simulink model "SYSTEM_MODEL"  (R2024a)
settings: Solver=ode45  StartTime=0.0  StopTime=0.5  RelTol=1e-3
values from neighbouring files (symbols this model uses):
  Cf = x*Cb    (= 0.000348151438014)    [parameters.m]
  Fsw = 10e3    (= 10000)    [parameters.m]
  kii = 219.7931    [parameters.m]
  kiv = 645.1962    [parameters.m]
  kpi = 4.9973    [parameters.m]
  kpv = 2.0537    [parameters.m]
  L = Vdc/(8*Fsw*I_ripple)    [parameters.m]
  Lf = L*r    [parameters.m]
  Lt = L+Lf    [parameters.m]
  R = 0.004    [parameters.m]
  Rf = 0.001    [parameters.m]
  Vdc = 800    [parameters.m]
undefined symbols (not defined in the file or in its folder): Ion, Lithium
libraries: spsIGBTDiodeLib x7, spsSeriesRLCBranchLib x5, slpidlib x5, spsCurrentMeasurementLib x3, spsVoltageMeasurementLib x3, spsThreePhaseSeriesRLCBranchLib x3, spsabctodq0Lib x2, simulink x1, spsIGBTLib x1, spsPWMGeneratorDCDCLib x1, spsBatteryLib x1, spsGroundLib x1
settings Model: Creator=devashishraj  LastModifiedBy=loran
settings DebuggingCC: UnconnectedInputMsg=warning  UnconnectedOutputMsg=warning  UnconnectedLineMsg=warning
settings ModelReferenceCC: EnableRefExpFcnMdlSchedulingChecks=on
settings RTWCC: GPUComputeCapability=3.5  DLArmComputeVersion=19.05

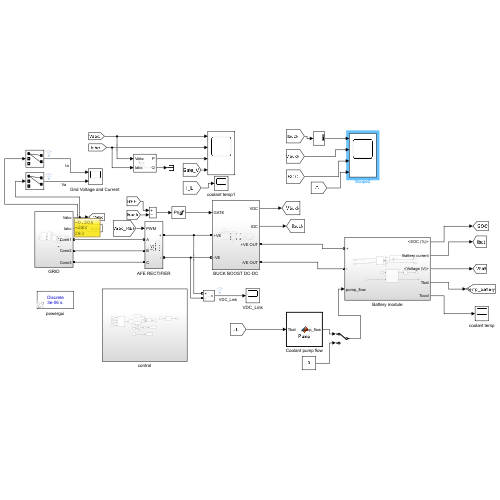
[thumbnail: Simulink's stored preview of the top-level diagram]
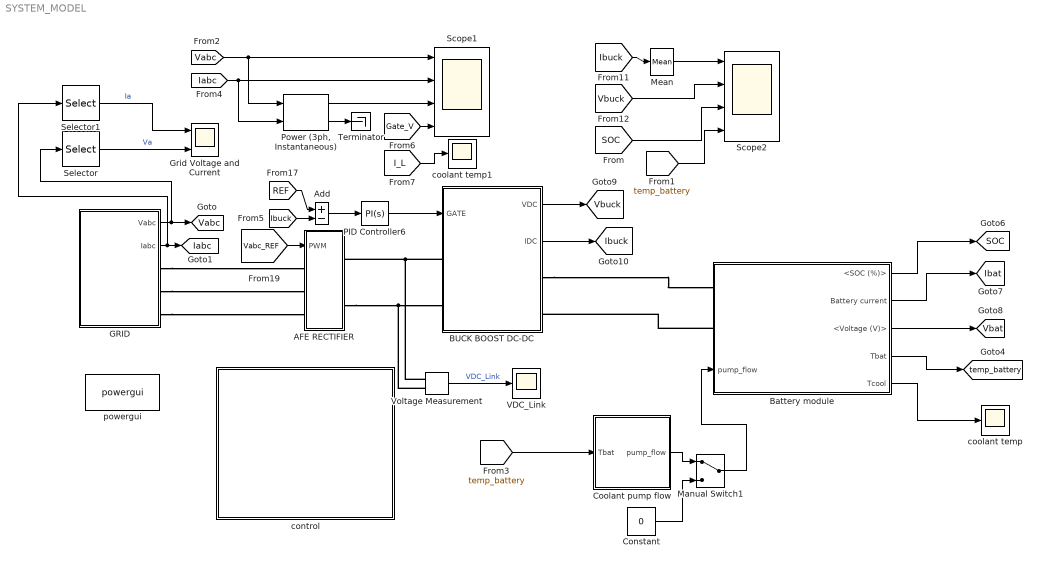
== system SYSTEM_MODEL ==
  AFE RECTIFIER : Subsystem
  Add : Sum  Inputs=+-
  BUCK BOOST DC-DC : Subsystem
  Battery module : Subsystem
      settings: PortSchema="{\"entries\":[{\"content\":{\"sides\":[{\"content\":{\"connectorIds\":[\"LConn1\",\"LConn2\",\"In1\"]},\"type\":\"ConnectorPlacement.EquallySpacedRectSide\",\"uuid\":\"b9a7e7ab-cfc6-4f27-ac3f-4a3ea86e3158\"},{\"content\":{\"connectorIds\":[\"Out1\",\"Out2\",\"Out3\",\"Out4\",\"Out5\"],\"side\":\"RIGHT\"},\"type\":\"ConnectorPlacement.EquallySpacedRectSide\",\"uuid\":\"900f3018-bf12-407b-85a8-bc4a87dc546d\"},{\"content\":{\"side\":\"TOP\"},\"type\":\"ConnectorPlacement.EquallySpacedRectSide\",\"uuid\":\"2d743f8c-64eb-4470-8afd-3ba3a990ea7c\"},{\"content\":{\"side\":\"BOTTOM\"},\"type\":\"ConnectorPlacement.EquallySpacedRectSide\",\"uuid\":\"3e69f90f-b07e-44a2-b438-8ead40159241\"}]},\"type\":\"ConnectorPlacement.EquallySpacedConnector\",\"uuid\":\"2127e1cc-c587-4944-bbda-621e2cf85e2c\"}],\"packageUris\":[\"http://schema.mathworks.com/mf0/Connector/R2020b\"],\"version\":\"1.0\"}"
  Constant : Constant  Value=0
  Coolant pump flow : MATLAB Function  TreatAsAtomicUnit=on
  GRID : Subsystem
  "Grid Voltage and Current " : Scope  NumInputPorts=2
  Manual Switch1 : ManualSwitch
  Mean : spsMeanLib/Mean  Freq=100  Vinit=0  Ts=0
  PID Controller6 : slpidlib/PID Controller  Controller=PI  Form=Parallel  TimeDomain=Continuous-time  UseExternalTs=off  SampleTime=-1  IntegratorMethod=Forward Euler  FilterMethod=Forward Euler  ControllerParametersSource=internal  P=800.07973079426302e-05  I=3.0202336655835159303  UseKiTs=off  D=0  UseExternalDerivativeSource=off  N=100  UseFilter=on  TunerSelectOption=Transfer Function Based (PID Tuner App)  ZeroCross=off  InitialConditionSource=internal  InitialConditionForIntegrator=0  InitialConditionForFilter=0  DifferentiatorICPrevScaledInput=0  ExternalReset=none  TrackingMode=off  Kt=1  LimitOutput=on  SatLimitsSource=internal  UpperSaturationLimit=0.47  LowerSaturationLimit=0  LinearizeAsGain=on  AntiWindupMode=clamping  Kb=1  LimitIntegrator=off  UpperIntegratorSaturationLimit=inf  LowerIntegratorSaturationLimit=-inf  POutMin=[]  POutMax=[]  IOutMin=[]  IOutMax=[]  DOutMin=[]  DOutMax=[]  NOutMin=[]  NOutMax=[]  SumOutMin=[]  SumOutMax=[]  SaturationOutMin=[]  SaturationOutMax=[]  PParamMin=[]  PParamMax=[]  IParamMin=[]  IParamMax=[]  DParamMin=[]  DParamMax=[]  NParamMin=[]  NParamMax=[]  KbParamMin=[]  KbParamMax=[]  KtParamMin=[]  KtParamMax=[]  KbOutMin=[]  KbOutMax=[]  KtOutMin=[]  KtOutMax=[]  IntegratorOutMin=[]  IntegratorOutMax=[]  FilterOutMin=[]  FilterOutMax=[]  SumI1OutMin=[]  SumI1OutMax=[]  SumI2OutMin=[]  SumI2OutMax=[]  SumI3OutMin=[]  SumI3OutMax=[]  SumI4OutMin=[]  SumI4OutMax=[]  SumDOutMin=[]  SumDOutMax=[]  DifferentiatorOutMin=[]  DifferentiatorOutMax=[]  FilterDiffOutCoefMin=[]  FilterDiffOutCoefMax=[]  ReciprocalOutMin=[]  ReciprocalOutMax=[]  SumDenOutMin=[]  SumDenOutMax=[]  SumNumOutMin=[]  SumNumOutMax=[]  DivideOutMin=[]  DivideOutMax=[]  UdiffTsProdOutMin=[]  UdiffTsProdOutMax=[]  NTsProdOutMin=[]  NTsProdOutMax=[]  UintegralTsProdOutMin=[]  UintegralTsProdOutMax=[]  UngainTsProdOutMin=[]  UngainTsProdOutMax=[]  ClampingZeroOutDataTypeStr=Inherit: Inherit via back propagation  ClampingZeroOutMin=[]  ClampingZeroOutMax=[]  FilterDenConstantOutDataTypeStr=Inherit: Inherit via back propagation  FilterDenConstantOutMin=[]  FilterDenConstantOutMax=[]  PCopyOutDataTypeStr=Inherit: Inherit via back propagation  PCopyOutMin=[]  PCopyOutMax=[]  NCopyOutDataTypeStr=Inherit: Inherit via back propagation  NCopyOutMin=[]  NCopyOutMax=[]  IntegratorContinuousStateAttributes=''  IntegratorStateMustResolveToSignalObject=off  IntegratorRTWStateStorageClass=Auto  FilterContinuousStateAttributes=''  FilterStateMustResolveToSignalObject=off  FilterRTWStateStorageClass=Auto  ParallelPVariant=InternalParameters  IdealPVariant=Disabled  IVariant=InternalParameters  DVariant=Disabled  IntegratorVariant=Continuous  SatVariant=Enabled  AWVariant=ContClampingParallel  PCopyVariant=Disabled  TRVariant=Disabled  FdbkBlocksVariant=Forward  IdealPFdbkVariant=Disabled  SatFdbkVariant=Disabled  DerivativeFilterVariant=Disabled  NVariant=Disabled  NCopyVariant=Disabled_SignalSpec  FilterICVariant=Disabled  IntegratorICVariant=InternalICs  ExternalResetVariant=Disabled  TRSumVariant=Passthrough  SumFdbkVariant=Disabled  SumVariant=Sum_PI  TsampFilterVariant=InternalTs  TsampNgainVariant=Passthrough  TsampIntegralVariant=Disabled_SignalSpec  ExternalSaturationOutDataTypeStr=Inherit: Same as second input  DerivativeSourceVariant=Disabled
  "Power (3ph, Instantaneous)" : spsPower3phInstantaneousLib/Power (3ph, Instantaneous)
  Scope1 : Scope  NumInputPorts=4
  Scope2 : Scope  NumInputPorts=4
  Selector : Selector  InputPortWidth=3  IndexOptions=Index vector (dialog)  Indices=[1 1]  OutputSizes=1
  Selector1 : Selector  InputPortWidth=3  IndexOptions=Index vector (dialog)  Indices=[1 1]  OutputSizes=1
  Terminator : Terminator
  VDC_Link : Scope
  Voltage Measurement : spsVoltageMeasurementLib/Voltage Measurement  PhasorSimulation=off  OutputType=Complex  PSBequivalent=0
  control : Subsystem
  coolant temp : Scope
  coolant temp1 : Scope
  powergui : spspowerguiLib/powergui  Priority=1  SimulationMode=Discrete  SampleTime=3e-6  frequency=60  Iterations=50  frequencyindice=0  Pbase=100e6  ErrMax=1e-4  UnitsV=kV  UnitsW=MW  buscounter=0  FunctionMessages=off  echomessages=off  EnableUseOfTLC=off  CurrentSourceSwitches=off  DisableSnubberDevices=off  DisableRonSwitches=off  DisableVfSwitches=off  DisplayEquations=off  AutomaticDiscreteSolvers=off  SolverType=Tustin/Backward Euler (TBE)  Interpol=off  ExternalGateDelay=off  methode=off  Ts=100  x0status=blocks  SPID=on  SwTol=0  HookPort=off  NonlinearTolerance=1e-4  nMaxIteration=100  ContinueOnMaxIteration=off  RestoreLinks=warning  ResistiveCurrentMeasurement=off  Frange=[0:2:500]  Ylog=off  Xlog=on  ShowGrid=off  save=off  variable=ZData  structure=0  ZoomFFT=off  StartTime=0.0  cycles=1  DisplayStyle=1  fundamental=60  FreqAxis=off  MaxFrequency=1000  frequencyindicesteady=1  RmsSteady=1  display=off
  tag scope: Iabc=global, Ibat=global, Ibuck=global, SOC=global, Vabc=global, Vbat=global, Vbuck=global, temp_battery=global
  wires:
  GRID/1(Vabc) -> Selector/1, [Vabc]
  GRID/2(Iabc) -> Selector1/1, [Iabc]
  [Ibuck] -> Add/2
  Add/1 -> PID Controller6/1
  [Ibuck] -> Mean/1
  [SOC] -> Scope2/3
  [REF] -> Add/1
  [Vabc_REF] -> AFE RECTIFIER/1(PWM)
  PID Controller6/1 -> BUCK BOOST DC-DC/1(GATE)
  BUCK BOOST DC-DC/1(VDC) -> [Vbuck]
  BUCK BOOST DC-DC/2(IDC) -> [Ibuck]
  [Vbuck] -> Scope2/2
  Mean/1 -> Scope2/1
  [temp_battery] -> Scope2/4
  Coolant pump flow/1(pump_flow) -> Manual Switch1/1
  Battery module/1(<SOC (%)>) -> [SOC]
  Battery module/2(Battery current) -> [Ibat]
  Battery module/3(<Voltage (V)>) -> [Vbat]
  Battery module/4(Tbat) -> [temp_battery]
  Battery module/5(Tcool) -> coolant temp/1
  Constant/1 -> Manual Switch1/2
  [temp_battery] -> Coolant pump flow/1(Tbat)
  Manual Switch1/1 -> Battery module/1(pump_flow)
  [Iabc] -> "Power (3ph, Instantaneous)"/2, Scope1/2
  [Vabc] -> "Power (3ph, Instantaneous)"/1, Scope1/1
  "Power (3ph, Instantaneous)"/1 -> Scope1/3
  [Gate_V] -> Scope1/4
  "Power (3ph, Instantaneous)"/2 -> Terminator/1
  [I_L] -> coolant temp1/1
  Selector1/1 -> "Grid Voltage and Current "/1  "Ia"
  Selector/1 -> "Grid Voltage and Current "/2  "Va"
  Voltage Measurement/1 -> VDC_Link/1  "VDC_Link"
  connections:
  GRID/RConn1 -- AFE RECTIFIER/LConn1
  GRID/RConn2 -- AFE RECTIFIER/LConn2
  GRID/RConn3 -- AFE RECTIFIER/LConn3
  BUCK BOOST DC-DC/LConn1 -- Voltage Measurement/LConn1 -- AFE RECTIFIER/RConn1
  AFE RECTIFIER/RConn2 -- Voltage Measurement/LConn2 -- BUCK BOOST DC-DC/LConn2
  BUCK BOOST DC-DC/RConn1 -- Battery module/LConn1
  Battery module/LConn2 -- BUCK BOOST DC-DC/RConn2

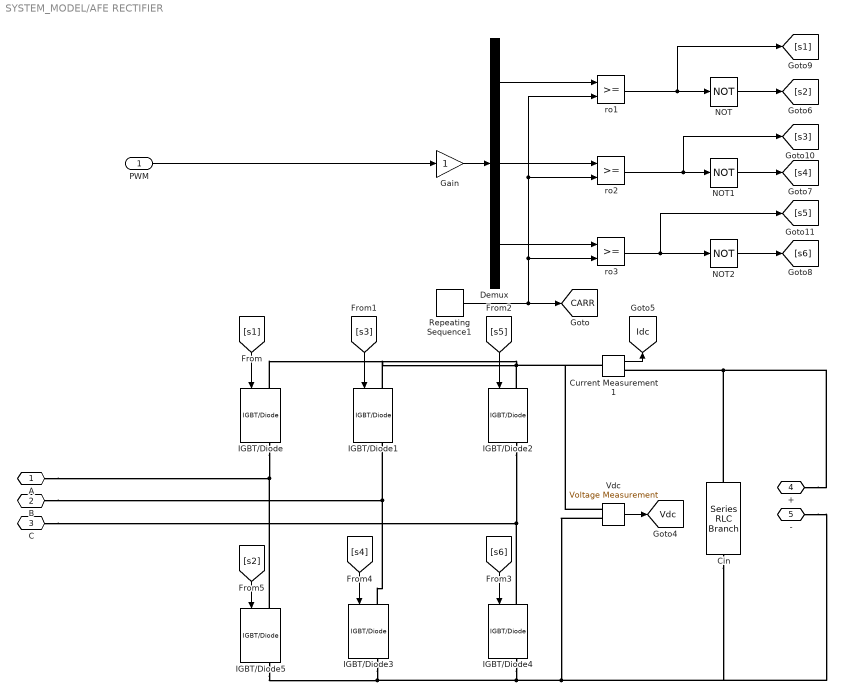
== system SYSTEM_MODEL/AFE RECTIFIER ==
  PWM : Inport
  Cin : spsSeriesRLCBranchLib/Series RLC Branch  LConnTagsString=__new0  RConnTagsString=__new0  BranchType=C  Resistance=1  Inductance=1e-3  SetiL0=off  InitialCurrent=0  Capacitance=1000e-6  Setx0=off  InitialVoltage=600  Measurements=None
  Current Measurement1 : spsCurrentMeasurementLib/Current Measurement  PhasorSimulation=off  OutputType=Complex  PSBequivalent=0
  Demux : Demux  Outputs=3
  Gain : Gain
  IGBT/Diode{,1..5} (6 alike) : spsIGBTDiodeLib/IGBT//Diode  Ron=1e-3  Rs=1e5  Cs=inf  Measurements=on
  NOT : Logic  Operator=NOT  IconShape=distinctive  AllPortsSameDT=off  OutDataTypeStr=boolean
  NOT1 : Logic  Operator=NOT  IconShape=distinctive  AllPortsSameDT=off  OutDataTypeStr=boolean
  NOT2 : Logic  Operator=NOT  IconShape=distinctive  AllPortsSameDT=off  OutDataTypeStr=boolean
  Repeating Sequence1 : simulink/Sources/Repeating Sequence  rep_seq_t="[0  1/(2*Fsw) 1/Fsw ]"  rep_seq_y=[-1000 1000 -1000]
  Vdc : spsVoltageMeasurementLib/Voltage Measurement  PhasorSimulation=off  OutputType=Complex  PSBequivalent=0
  ro1 : RelationalOperator  OutDataTypeStr=boolean  RndMeth=Simplest  InputSameDT=off
  ro2 : RelationalOperator  OutDataTypeStr=boolean  RndMeth=Simplest  InputSameDT=off
  ro3 : RelationalOperator  OutDataTypeStr=boolean  RndMeth=Simplest  InputSameDT=off
  A : PMIOPort  Side=Left
  B : PMIOPort  Port=2  Side=Left
  C : PMIOPort  Port=3  Side=Left
  + : PMIOPort  Port=4  Side=Right
  - : PMIOPort  Port=5  Side=Right
  tag scope: CARR=global, Idc=global, Vdc=global
  wires:
  NOT2/1 -> [s6]
  Demux/2 -> ro2/1
  PWM/1 -> Gain/1
  [s3] -> IGBT/Diode1/1
  Current Measurement1/1 -> [Idc]
  [s1] -> IGBT/Diode/1
  [s4] -> IGBT/Diode3/1
  Gain/1 -> Demux/1
  Demux/1 -> ro1/1
  [s2] -> IGBT/Diode5/1
  [s5] -> IGBT/Diode2/1
  ro1/1 -> [s1], NOT/1
  ro2/1 -> [s3], NOT1/1
  Demux/3 -> ro3/1
  NOT1/1 -> [s4]
  NOT/1 -> [s2]
  [s6] -> IGBT/Diode4/1
  Vdc/1 -> [Vdc]
  ro3/1 -> [s5], NOT2/1
  Repeating Sequence1/1 -> ro3/2, ro2/2, ro1/2, [CARR]
  connections:
  C/RConn1 -- IGBT/Diode4/LConn1 -- IGBT/Diode2/RConn1
  -/RConn1 -- Cin/RConn1 -- Vdc/LConn2 -- IGBT/Diode5/RConn1 -- IGBT/Diode3/RConn1 -- IGBT/Diode4/RConn1
  Cin/LConn1 -- +/RConn1 -- Current Measurement1/RConn1
  Vdc/LConn1 -- Current Measurement1/LConn1 -- IGBT/Diode2/LConn1 -- IGBT/Diode/LConn1 -- IGBT/Diode1/LConn1
  B/RConn1 -- IGBT/Diode3/LConn1 -- IGBT/Diode1/RConn1
  A/RConn1 -- IGBT/Diode5/LConn1 -- IGBT/Diode/RConn1

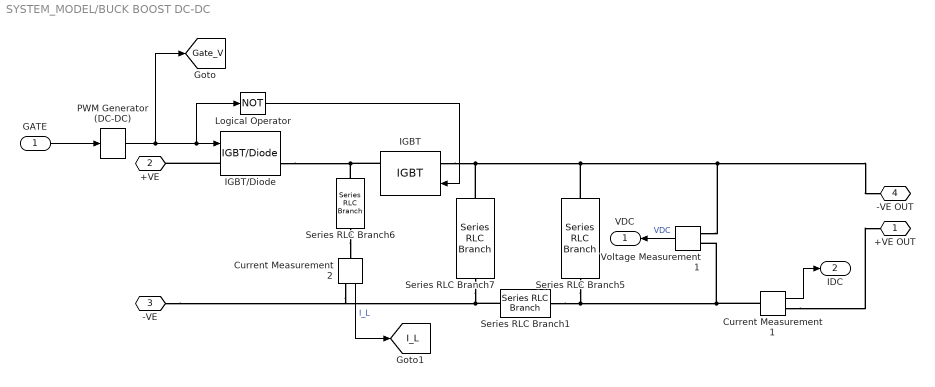
== system SYSTEM_MODEL/BUCK BOOST DC-DC ==
  GATE : Inport
  Current Measurement1 : spsCurrentMeasurementLib/Current Measurement  PhasorSimulation=off  OutputType=Complex  PSBequivalent=0
  Current Measurement2 : spsCurrentMeasurementLib/Current Measurement  PhasorSimulation=off  OutputType=Complex  PSBequivalent=0
  IGBT : spsIGBTLib/IGBT  Ron=0.001  Lon=0  Vf=1  Tf=1e-6  Tt=2e-6  IC=0  Rs=1e5  Cs=inf  Measurements=on
  IGBT/Diode : spsIGBTDiodeLib/IGBT//Diode  Ron=1e-3  Rs=1e5  Cs=inf  Measurements=on
  Logical Operator : Logic  Operator=NOT  AllPortsSameDT=off  OutDataTypeStr=boolean
  PWM Generator (DC-DC) : spsPWMGeneratorDCDCLib/PWM Generator (DC-DC)  Fsw=100e3  Ts=0
  Series RLC Branch1 : spsSeriesRLCBranchLib/Series RLC Branch  LConnTagsString=__new0  RConnTagsString=__new0  BranchType=L  Resistance=1  Inductance=3e-3  SetiL0=on  InitialCurrent=0  Capacitance=1e-6  Setx0=off  InitialVoltage=0  Measurements=Branch current
  Series RLC Branch5 : spsSeriesRLCBranchLib/Series RLC Branch  LConnTagsString=__new0  RConnTagsString=__new0  BranchType=C  Resistance=1  Inductance=1e-3  SetiL0=off  InitialCurrent=0  Capacitance=500e-6  Setx0=on  InitialVoltage=0  Measurements=None
  Series RLC Branch6 : spsSeriesRLCBranchLib/Series RLC Branch  LConnTagsString=__new0  RConnTagsString=__new0  BranchType=L  Resistance=1  Inductance=36e-6  SetiL0=on  InitialCurrent=0  Capacitance=1e-6  Setx0=off  InitialVoltage=0  Measurements=Branch current
  Series RLC Branch7 : spsSeriesRLCBranchLib/Series RLC Branch  LConnTagsString=__new0  RConnTagsString=__new0  BranchType=C  Resistance=1  Inductance=1e-3  SetiL0=off  InitialCurrent=0  Capacitance=20e-6  Setx0=on  InitialVoltage=0  Measurements=None
  Voltage Measurement1 : spsVoltageMeasurementLib/Voltage Measurement  PhasorSimulation=off  OutputType=Complex  PSBequivalent=0
  +VE OUT : PMIOPort  Side=Right
  +VE : PMIOPort  Port=2  Side=Left
  -VE : PMIOPort  Port=3  Side=Left
  -VE OUT : PMIOPort  Port=4  Side=Right
  VDC : Outport
  IDC : Outport  Port=2
  tag scope: Gate_V=global, I_L=global
  wires:
  Logical Operator/1 -> IGBT/1
  Current Measurement1/1 -> IDC/1
  GATE/1 -> PWM Generator (DC-DC)/1
  PWM Generator (DC-DC)/1 -> [Gate_V], IGBT/Diode/1, Logical Operator/1
  Voltage Measurement1/1 -> VDC/1  "VDC"
  Current Measurement2/1 -> [I_L]  "I_L"
  connections:
  IGBT/LConn1 -- Series RLC Branch7/RConn1 -- Series RLC Branch5/RConn1 -- -VE OUT/RConn1 -- Voltage Measurement1/LConn2
  Series RLC Branch5/LConn1 -- Series RLC Branch1/RConn1 -- Voltage Measurement1/LConn1 -- Current Measurement1/LConn1
  Series RLC Branch1/LConn1 -- -VE/RConn1 -- Current Measurement2/RConn1 -- Series RLC Branch7/LConn1
  IGBT/RConn1 -- Series RLC Branch6/RConn1 -- IGBT/Diode/RConn1
  IGBT/Diode/LConn1 -- +VE/RConn1
  Current Measurement1/RConn1 -- +VE OUT/RConn1
  Series RLC Branch6/LConn1 -- Current Measurement2/LConn1

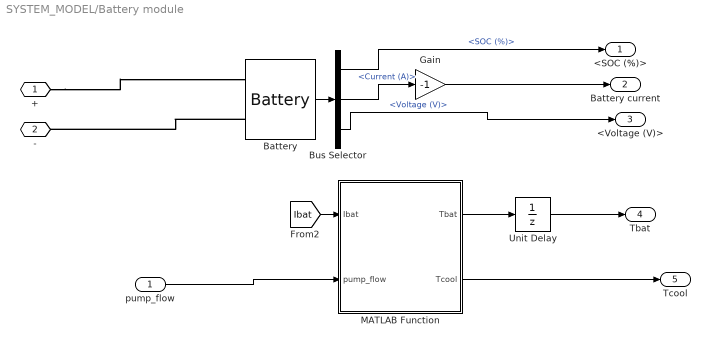
== system SYSTEM_MODEL/Battery module ==
  pump_flow : Inport
  Battery : spsBatteryLib/Battery  BatType=Lithium-Ion  ShowTempParam=off  ThermalPreset=no  ShowAgeParam=off  NomV=400  NomQ=250  SOC=20  Batt_Tr=1  PresetModel=on  MaxQ=250  MinV=300  FullV=465.5949  Dis_rate=108.6957  R=0.016  Normal_OP=226.087  expZone="[432.1543      12.28261]"  current=[6.5 13 32.5]  Units=Time  Tci=25  NomT=25  T2=20  MaxQ2=250  FullV2=400  Normal_OP2=440  expZone2=[450 250]  Rca=0.6  ti=2000  Dp=0  Neq0=0  Tsim=1e6  Ta1=25  Qeol=5.4*0.9  Reol=0.013333*1.2  Char_age=[2.3478, 3]  Dis_age=[2.3478, 10]  N1=1500  N2=10500  N3=1000  N4=1400  Ta2=45  N5=950
  Bus Selector : BusSelector  OutputSignals=SOC (%),Current (A),Voltage (V)
  Gain : Gain  Gain=-1
  MATLAB Function : MATLAB Function  TreatAsAtomicUnit=on
  Unit Delay : UnitDelay  SampleTime=-1  HasFrameUpgradeWarning=on
  + : PMIOPort  Side=Left
  - : PMIOPort  Port=2  Side=Left
  <SOC (%)> : Outport
  Battery current : Outport  Port=2
  <Voltage (V)> : Outport  Port=3
  Tbat : Outport  Port=4
  Tcool : Outport  Port=5
  wires:
  MATLAB Function/2(Tcool) -> Tcool/1
  Bus Selector/1 -> <SOC (%)>/1  "<SOC (%)>"
  Battery/1 -> Bus Selector/1
  [Ibat] -> MATLAB Function/1(Ibat)
  Bus Selector/2 -> Gain/1  "<Current (A)>"
  pump_flow/1 -> MATLAB Function/2(pump_flow)
  Bus Selector/3 -> <Voltage (V)>/1  "<Voltage (V)>"
  MATLAB Function/1(Tbat) -> Unit Delay/1
  Gain/1 -> Battery current/1
  Unit Delay/1 -> Tbat/1
  connections:
  Battery/LConn2 -- -/RConn1
  +/RConn1 -- Battery/LConn1

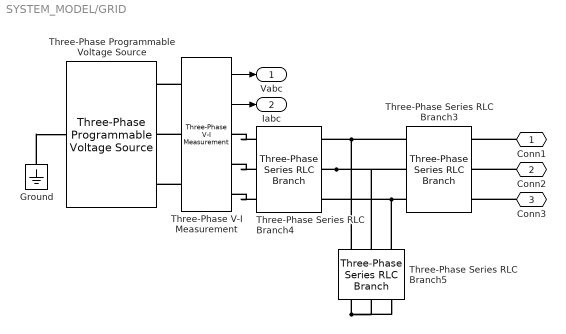
== system SYSTEM_MODEL/GRID ==
  Ground : spsGroundLib/Ground  LConnTagsString=a
  Three-Phase Programmable Voltage Source : spsThreePhaseProgrammableVoltageSourceLib/Three-Phase Programmable Voltage Source  PositiveSequence="[400  0 50]"  VariationEntity=None  VariationType=Table of time-amplitude pairs  VariationTypeAlt=Step  VariationStep=0.5  VariationRate=10  VariationMagnitude=0.3  VariationFrequency=2  VariationTiming=[1 2]  VariationPhaseA=off  Amplitudes=[1 0.8 1.2 1.0]  TimeValues=[0 0.1 0.15 0.2]  HarmonicGeneration=off  HarmonicA=[3 0.2 -25 0]  HarmonicB=[2 0.15 35 2]  Timing="[0.05  3]"  BusType=swing  Pref=0  Qref=0  Qmin=-inf  Qmax=inf
  Three-Phase Series RLC Branch3 : spsThreePhaseSeriesRLCBranchLib/Three-Phase Series RLC Branch  LConnTagsString=A|B|C  RConnTagsString=A|B|C  BranchType=RL  Resistance=R  Inductance=L  Capacitance=1e-6  Measurements=None
  Three-Phase Series RLC Branch4 : spsThreePhaseSeriesRLCBranchLib/Three-Phase Series RLC Branch  LConnTagsString=A|B|C  RConnTagsString=A|B|C  BranchType=RL  Resistance=Rf  Inductance=Lf  Capacitance=1e-6  Measurements=None
  Three-Phase Series RLC Branch5 : spsThreePhaseSeriesRLCBranchLib/Three-Phase Series RLC Branch  LConnTagsString=A|B|C  RConnTagsString=A|B|C  BranchType=RC  Resistance=2  Inductance=150e-6  Capacitance=Cf  Measurements=None
  Three-Phase V-I Measurement : spsThreePhaseVIMeasurementLib/Three-Phase V-I Measurement  VoltageMeasurement=phase-to-ground  SetLabelV=off  LabelV=Vabc  Vpu=off  VpuLL=off  CurrentMeasurement=yes  SetLabelI=off  LabelI=Iabc  Ipu=off  Pbase=100e6  Vbase=500e3  OutputType=Complex  PhasorSimulation=off  PSBequivalent=0
  Conn1 : PMIOPort  Side=Right
  Conn2 : PMIOPort  Port=2  Side=Right
  Conn3 : PMIOPort  Port=3  Side=Right
  Vabc : Outport
  Iabc : Outport  Port=2
  wires:
  Three-Phase V-I Measurement/1 -> Vabc/1
  Three-Phase V-I Measurement/2 -> Iabc/1
  connections:
  Three-Phase V-I Measurement/LConn1 -- Three-Phase Programmable Voltage Source/RConn1
  Three-Phase V-I Measurement/LConn3 -- Three-Phase Programmable Voltage Source/RConn3
  Three-Phase V-I Measurement/LConn2 -- Three-Phase Programmable Voltage Source/RConn2
  Ground/LConn1 -- Three-Phase Programmable Voltage Source/LConn1
  Three-Phase Series RLC Branch4/LConn2 -- Three-Phase Series RLC Branch5/LConn2 -- Three-Phase Series RLC Branch3/RConn2
  Three-Phase Series RLC Branch3/RConn3 -- Three-Phase Series RLC Branch4/LConn3 -- Three-Phase Series RLC Branch5/LConn3
  Three-Phase Series RLC Branch5/LConn1 -- Three-Phase Series RLC Branch4/LConn1 -- Three-Phase Series RLC Branch3/RConn1
  Three-Phase Series RLC Branch5/RConn1 -- Three-Phase Series RLC Branch5/RConn2 -- Three-Phase Series RLC Branch5/RConn3
  Conn3/RConn1 -- Three-Phase Series RLC Branch3/LConn3
  Conn1/RConn1 -- Three-Phase Series RLC Branch3/LConn1
  Conn2/RConn1 -- Three-Phase Series RLC Branch3/LConn2
  Three-Phase Series RLC Branch4/RConn1 -- Three-Phase V-I Measurement/RConn1
  Three-Phase Series RLC Branch4/RConn2 -- Three-Phase V-I Measurement/RConn2
  Three-Phase Series RLC Branch4/RConn3 -- Three-Phase V-I Measurement/RConn3

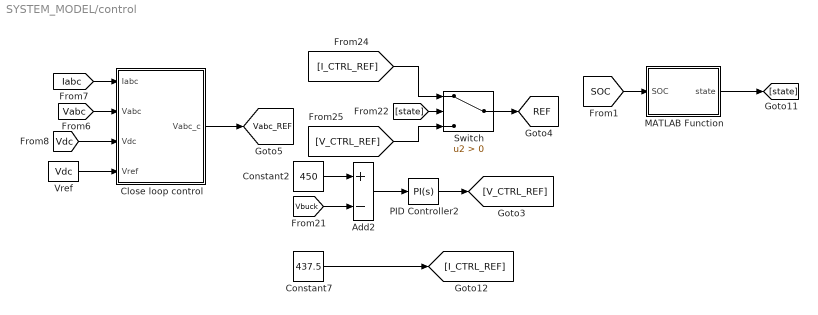
== system SYSTEM_MODEL/control ==
  Add2 : Sum  Inputs=+-
  Close loop control : Subsystem
  Constant2 : Constant  Value=450  SampleTime=2e-6
  Constant7 : Constant  Value=437.5  SampleTime=2e-6
  MATLAB Function : MATLAB Function  TreatAsAtomicUnit=on
  PID Controller2 : slpidlib/PID Controller  Controller=PI  Form=Parallel  TimeDomain=Continuous-time  UseExternalTs=off  SampleTime=-1  IntegratorMethod=Forward Euler  FilterMethod=Forward Euler  ControllerParametersSource=internal  P=0.75  I=50  UseKiTs=off  D=0  UseExternalDerivativeSource=off  N=100  UseFilter=on  TunerSelectOption=Transfer Function Based (PID Tuner App)  ZeroCross=off  InitialConditionSource=internal  InitialConditionForIntegrator=0  InitialConditionForFilter=0  DifferentiatorICPrevScaledInput=0  ExternalReset=none  TrackingMode=off  Kt=1  LimitOutput=on  SatLimitsSource=internal  UpperSaturationLimit=500  LowerSaturationLimit=0  LinearizeAsGain=on  AntiWindupMode=clamping  Kb=1  LimitIntegrator=off  UpperIntegratorSaturationLimit=inf  LowerIntegratorSaturationLimit=-inf  POutMin=[]  POutMax=[]  IOutMin=[]  IOutMax=[]  DOutMin=[]  DOutMax=[]  NOutMin=[]  NOutMax=[]  SumOutMin=[]  SumOutMax=[]  SaturationOutMin=[]  SaturationOutMax=[]  PParamMin=[]  PParamMax=[]  IParamMin=[]  IParamMax=[]  DParamMin=[]  DParamMax=[]  NParamMin=[]  NParamMax=[]  KbParamMin=[]  KbParamMax=[]  KtParamMin=[]  KtParamMax=[]  KbOutMin=[]  KbOutMax=[]  KtOutMin=[]  KtOutMax=[]  IntegratorOutMin=[]  IntegratorOutMax=[]  FilterOutMin=[]  FilterOutMax=[]  SumI1OutMin=[]  SumI1OutMax=[]  SumI2OutMin=[]  SumI2OutMax=[]  SumI3OutMin=[]  SumI3OutMax=[]  SumI4OutMin=[]  SumI4OutMax=[]  SumDOutMin=[]  SumDOutMax=[]  DifferentiatorOutMin=[]  DifferentiatorOutMax=[]  FilterDiffOutCoefMin=[]  FilterDiffOutCoefMax=[]  ReciprocalOutMin=[]  ReciprocalOutMax=[]  SumDenOutMin=[]  SumDenOutMax=[]  SumNumOutMin=[]  SumNumOutMax=[]  DivideOutMin=[]  DivideOutMax=[]  UdiffTsProdOutMin=[]  UdiffTsProdOutMax=[]  NTsProdOutMin=[]  NTsProdOutMax=[]  UintegralTsProdOutMin=[]  UintegralTsProdOutMax=[]  UngainTsProdOutMin=[]  UngainTsProdOutMax=[]  ClampingZeroOutDataTypeStr=Inherit: Inherit via back propagation  ClampingZeroOutMin=[]  ClampingZeroOutMax=[]  FilterDenConstantOutDataTypeStr=Inherit: Inherit via back propagation  FilterDenConstantOutMin=[]  FilterDenConstantOutMax=[]  PCopyOutDataTypeStr=Inherit: Inherit via back propagation  PCopyOutMin=[]  PCopyOutMax=[]  NCopyOutDataTypeStr=Inherit: Inherit via back propagation  NCopyOutMin=[]  NCopyOutMax=[]  IntegratorContinuousStateAttributes=''  IntegratorStateMustResolveToSignalObject=off  IntegratorRTWStateStorageClass=Auto  FilterContinuousStateAttributes=''  FilterStateMustResolveToSignalObject=off  FilterRTWStateStorageClass=Auto  ParallelPVariant=InternalParameters  IdealPVariant=Disabled  IVariant=InternalParameters  DVariant=Disabled  IntegratorVariant=Continuous  SatVariant=Enabled  AWVariant=ContClampingParallel  PCopyVariant=Disabled  TRVariant=Disabled  FdbkBlocksVariant=Forward  IdealPFdbkVariant=Disabled  SatFdbkVariant=Disabled  DerivativeFilterVariant=Disabled  NVariant=Disabled  NCopyVariant=Disabled_SignalSpec  FilterICVariant=Disabled  IntegratorICVariant=InternalICs  ExternalResetVariant=Disabled  TRSumVariant=Passthrough  SumFdbkVariant=Disabled  SumVariant=Sum_PI  TsampFilterVariant=InternalTs  TsampNgainVariant=Passthrough  TsampIntegralVariant=Disabled_SignalSpec  ExternalSaturationOutDataTypeStr=Inherit: Same as second input  DerivativeSourceVariant=Disabled
  Switch : Switch  Criteria=u2 > Threshold  SaturateOnIntegerOverflow=off  InputSameDT=off
  Vref : Constant  Value=Vdc
  tag scope: REF=global, Vabc_REF=global
  wires:
  Close loop control/1(Vabc_c) -> [Vabc_REF]
  [Vdc] -> Close loop control/3(Vdc)
  MATLAB Function/1(state) -> [state]
  Add2/1 -> PID Controller2/1
  [SOC] -> MATLAB Function/1(SOC)
  [I_CTRL_REF] -> Switch/1
  Constant2/1 -> Add2/1
  PID Controller2/1 -> [V_CTRL_REF]
  [state] -> Switch/2
  [V_CTRL_REF] -> Switch/3
  Constant7/1 -> [I_CTRL_REF]
  [Vbuck] -> Add2/2
  Vref/1 -> Close loop control/4(Vref)
  [Iabc] -> Close loop control/1(Iabc)
  Switch/1 -> [REF]
  [Vabc] -> Close loop control/2(Vabc)

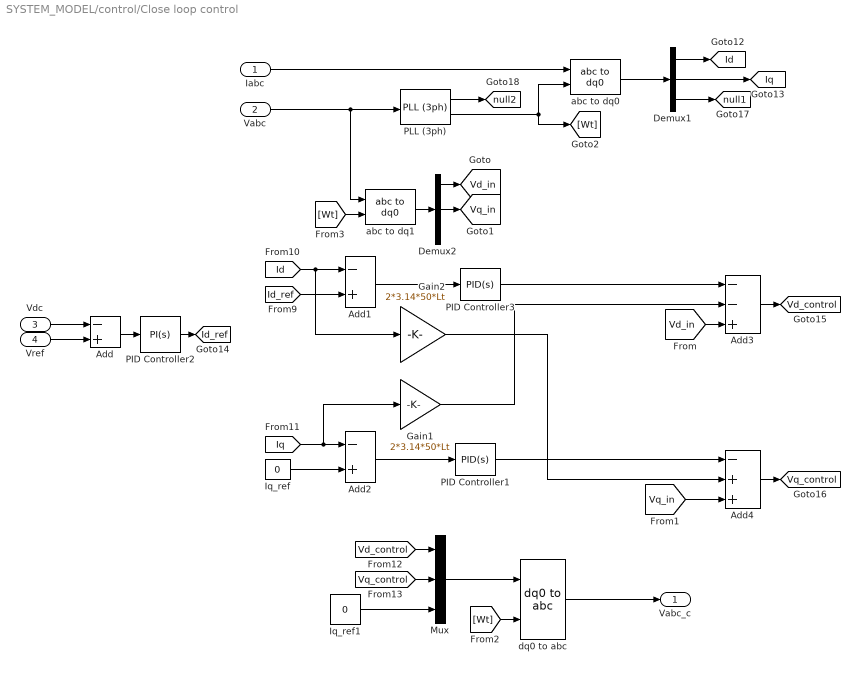
== system SYSTEM_MODEL/control/Close loop control ==
  Iabc : Inport
  Vabc : Inport  Port=2
  Vdc : Inport  Port=3
  Vref : Inport  Port=4
  Add : Sum  Inputs=-+
  Add1 : Sum  Inputs=-+
  Add2 : Sum  Inputs=-+
  Add3 : Sum  Inputs=--+
  Add4 : Sum  Inputs=-++
  Demux1 : Demux  Outputs=3
  Demux2 : Demux  Outputs=3
  Gain1 : Gain  Gain=2*3.14*50*Lt
  Gain2 : Gain  Gain=2*3.14*50*Lt
  Iq_ref : Constant  Value=0
  Iq_ref1 : Constant  Value=0
  Mux : Mux  Inputs=3
  PID Controller1 : slpidlib/PID Controller  Controller=PID  Form=Parallel  TimeDomain=Continuous-time  UseExternalTs=off  SampleTime=-1  IntegratorMethod=Forward Euler  FilterMethod=Forward Euler  ControllerParametersSource=internal  P=kpi  I=kii  UseKiTs=off  D=0  UseExternalDerivativeSource=off  N=100  UseFilter=on  TunerSelectOption=Transfer Function Based (PID Tuner App)  InitialConditionSource=internal  InitialConditionForIntegrator=0  InitialConditionForFilter=0  DifferentiatorICPrevScaledInput=0  ExternalReset=none  TrackingMode=off  Kt=1  LimitOutput=off  SatLimitsSource=internal  UpperSaturationLimit=inf  LowerSaturationLimit=-inf  LinearizeAsGain=on  AntiWindupMode=none  Kb=1  LimitIntegrator=off  UpperIntegratorSaturationLimit=inf  LowerIntegratorSaturationLimit=-inf  POutMin=[]  POutMax=[]  IOutMin=[]  IOutMax=[]  DOutMin=[]  DOutMax=[]  NOutMin=[]  NOutMax=[]  SumOutMin=[]  SumOutMax=[]  SaturationOutMin=[]  SaturationOutMax=[]  PParamMin=[]  PParamMax=[]  IParamMin=[]  IParamMax=[]  DParamMin=[]  DParamMax=[]  NParamMin=[]  NParamMax=[]  KbParamMin=[]  KbParamMax=[]  KtParamMin=[]  KtParamMax=[]  KbOutMin=[]  KbOutMax=[]  KtOutMin=[]  KtOutMax=[]  IntegratorOutMin=[]  IntegratorOutMax=[]  FilterOutMin=[]  FilterOutMax=[]  SumI1OutMin=[]  SumI1OutMax=[]  SumI2OutMin=[]  SumI2OutMax=[]  SumI3OutMin=[]  SumI3OutMax=[]  SumI4OutMin=[]  SumI4OutMax=[]  SumDOutMin=[]  SumDOutMax=[]  DifferentiatorOutMin=[]  DifferentiatorOutMax=[]  FilterDiffOutCoefMin=[]  FilterDiffOutCoefMax=[]  ReciprocalOutMin=[]  ReciprocalOutMax=[]  SumDenOutMin=[]  SumDenOutMax=[]  SumNumOutMin=[]  SumNumOutMax=[]  DivideOutMin=[]  DivideOutMax=[]  UdiffTsProdOutMin=[]  UdiffTsProdOutMax=[]  NTsProdOutMin=[]  NTsProdOutMax=[]  UintegralTsProdOutMin=[]  UintegralTsProdOutMax=[]  UngainTsProdOutMin=[]  UngainTsProdOutMax=[]  ClampingZeroOutDataTypeStr=Inherit: Inherit via back propagation  ClampingZeroOutMin=[]  ClampingZeroOutMax=[]  FilterDenConstantOutDataTypeStr=Inherit: Inherit via back propagation  FilterDenConstantOutMin=[]  FilterDenConstantOutMax=[]  PCopyOutDataTypeStr=Inherit: Inherit via back propagation  PCopyOutMin=[]  PCopyOutMax=[]  NCopyOutDataTypeStr=Inherit: Inherit via back propagation  NCopyOutMin=[]  NCopyOutMax=[]  IntegratorContinuousStateAttributes=''  IntegratorStateMustResolveToSignalObject=off  IntegratorRTWStateStorageClass=Auto  FilterContinuousStateAttributes=''  FilterStateMustResolveToSignalObject=off  FilterRTWStateStorageClass=Auto  ParallelPVariant=InternalParameters  IdealPVariant=Disabled  IVariant=InternalParameters  DVariant=InternalParameters  IntegratorVariant=Continuous  SatVariant=Disabled  AWVariant=Passthrough  PCopyVariant=Disabled  TRVariant=Disabled  FdbkBlocksVariant=Forward  IdealPFdbkVariant=Disabled  SatFdbkVariant=Disabled  DerivativeFilterVariant=ContFilter  NVariant=InternalParameters  NCopyVariant=Disabled  FilterICVariant=InternalICsFilter  IntegratorICVariant=InternalICs  ExternalResetVariant=Disabled  TRSumVariant=Passthrough  SumFdbkVariant=Disabled  SumVariant=Sum_PID  TsampFilterVariant=InternalTs  TsampNgainVariant=Passthrough  TsampIntegralVariant=Disabled_SignalSpec  ExternalSaturationOutDataTypeStr=Inherit: Same as second input  DerivativeSourceVariant=ErrorSignal
  PID Controller2 : slpidlib/PID Controller  Controller=PI  Form=Parallel  TimeDomain=Continuous-time  UseExternalTs=off  SampleTime=2e-6  IntegratorMethod=Forward Euler  FilterMethod=Forward Euler  ControllerParametersSource=internal  P=kpv  I=kiv  UseKiTs=off  D=0  UseExternalDerivativeSource=off  N=100  UseFilter=on  TunerSelectOption=Transfer Function Based (PID Tuner App)  InitialConditionSource=internal  InitialConditionForIntegrator=0  InitialConditionForFilter=0  DifferentiatorICPrevScaledInput=0  ExternalReset=none  TrackingMode=off  Kt=1  LimitOutput=off  SatLimitsSource=internal  UpperSaturationLimit=inf  LowerSaturationLimit=-inf  LinearizeAsGain=on  AntiWindupMode=none  Kb=1  LimitIntegrator=off  UpperIntegratorSaturationLimit=inf  LowerIntegratorSaturationLimit=-inf  POutMin=[]  POutMax=[]  IOutMin=[]  IOutMax=[]  DOutMin=[]  DOutMax=[]  NOutMin=[]  NOutMax=[]  SumOutMin=[]  SumOutMax=[]  SaturationOutMin=[]  SaturationOutMax=[]  PParamMin=[]  PParamMax=[]  IParamMin=[]  IParamMax=[]  DParamMin=[]  DParamMax=[]  NParamMin=[]  NParamMax=[]  KbParamMin=[]  KbParamMax=[]  KtParamMin=[]  KtParamMax=[]  KbOutMin=[]  KbOutMax=[]  KtOutMin=[]  KtOutMax=[]  IntegratorOutMin=[]  IntegratorOutMax=[]  FilterOutMin=[]  FilterOutMax=[]  SumI1OutMin=[]  SumI1OutMax=[]  SumI2OutMin=[]  SumI2OutMax=[]  SumI3OutMin=[]  SumI3OutMax=[]  SumI4OutMin=[]  SumI4OutMax=[]  SumDOutMin=[]  SumDOutMax=[]  DifferentiatorOutMin=[]  DifferentiatorOutMax=[]  FilterDiffOutCoefMin=[]  FilterDiffOutCoefMax=[]  ReciprocalOutMin=[]  ReciprocalOutMax=[]  SumDenOutMin=[]  SumDenOutMax=[]  SumNumOutMin=[]  SumNumOutMax=[]  DivideOutMin=[]  DivideOutMax=[]  UdiffTsProdOutMin=[]  UdiffTsProdOutMax=[]  NTsProdOutMin=[]  NTsProdOutMax=[]  UintegralTsProdOutMin=[]  UintegralTsProdOutMax=[]  UngainTsProdOutMin=[]  UngainTsProdOutMax=[]  ClampingZeroOutDataTypeStr=Inherit: Inherit via back propagation  ClampingZeroOutMin=[]  ClampingZeroOutMax=[]  FilterDenConstantOutDataTypeStr=Inherit: Inherit via back propagation  FilterDenConstantOutMin=[]  FilterDenConstantOutMax=[]  PCopyOutDataTypeStr=Inherit: Inherit via back propagation  PCopyOutMin=[]  PCopyOutMax=[]  NCopyOutDataTypeStr=Inherit: Inherit via back propagation  NCopyOutMin=[]  NCopyOutMax=[]  IntegratorContinuousStateAttributes=''  IntegratorStateMustResolveToSignalObject=off  IntegratorRTWStateStorageClass=Auto  FilterContinuousStateAttributes=''  FilterStateMustResolveToSignalObject=off  FilterRTWStateStorageClass=Auto  ParallelPVariant=InternalParameters  IdealPVariant=Disabled  IVariant=InternalParameters  DVariant=Disabled  IntegratorVariant=Continuous  SatVariant=Disabled  AWVariant=Passthrough  PCopyVariant=Disabled  TRVariant=Disabled  FdbkBlocksVariant=Forward  IdealPFdbkVariant=Disabled  SatFdbkVariant=Disabled  DerivativeFilterVariant=Disabled  NVariant=Disabled  NCopyVariant=Disabled_SignalSpec  FilterICVariant=Disabled  IntegratorICVariant=InternalICs  ExternalResetVariant=Disabled  TRSumVariant=Passthrough  SumFdbkVariant=Disabled  SumVariant=Sum_PI  TsampFilterVariant=InternalTs  TsampNgainVariant=Passthrough  TsampIntegralVariant=Disabled_SignalSpec  ExternalSaturationOutDataTypeStr=Inherit: Same as second input  DerivativeSourceVariant=Disabled
  PID Controller3 : slpidlib/PID Controller  Controller=PID  Form=Parallel  TimeDomain=Continuous-time  UseExternalTs=off  SampleTime=-1  IntegratorMethod=Forward Euler  FilterMethod=Forward Euler  ControllerParametersSource=internal  P=kpi  I=kii  UseKiTs=off  D=0  UseExternalDerivativeSource=off  N=100  UseFilter=on  TunerSelectOption=Transfer Function Based (PID Tuner App)  InitialConditionSource=internal  InitialConditionForIntegrator=0  InitialConditionForFilter=0  DifferentiatorICPrevScaledInput=0  ExternalReset=none  TrackingMode=off  Kt=1  LimitOutput=off  SatLimitsSource=internal  UpperSaturationLimit=inf  LowerSaturationLimit=-inf  LinearizeAsGain=on  AntiWindupMode=none  Kb=1  LimitIntegrator=off  UpperIntegratorSaturationLimit=inf  LowerIntegratorSaturationLimit=-inf  POutMin=[]  POutMax=[]  IOutMin=[]  IOutMax=[]  DOutMin=[]  DOutMax=[]  NOutMin=[]  NOutMax=[]  SumOutMin=[]  SumOutMax=[]  SaturationOutMin=[]  SaturationOutMax=[]  PParamMin=[]  PParamMax=[]  IParamMin=[]  IParamMax=[]  DParamMin=[]  DParamMax=[]  NParamMin=[]  NParamMax=[]  KbParamMin=[]  KbParamMax=[]  KtParamMin=[]  KtParamMax=[]  KbOutMin=[]  KbOutMax=[]  KtOutMin=[]  KtOutMax=[]  IntegratorOutMin=[]  IntegratorOutMax=[]  FilterOutMin=[]  FilterOutMax=[]  SumI1OutMin=[]  SumI1OutMax=[]  SumI2OutMin=[]  SumI2OutMax=[]  SumI3OutMin=[]  SumI3OutMax=[]  SumI4OutMin=[]  SumI4OutMax=[]  SumDOutMin=[]  SumDOutMax=[]  DifferentiatorOutMin=[]  DifferentiatorOutMax=[]  FilterDiffOutCoefMin=[]  FilterDiffOutCoefMax=[]  ReciprocalOutMin=[]  ReciprocalOutMax=[]  SumDenOutMin=[]  SumDenOutMax=[]  SumNumOutMin=[]  SumNumOutMax=[]  DivideOutMin=[]  DivideOutMax=[]  UdiffTsProdOutMin=[]  UdiffTsProdOutMax=[]  NTsProdOutMin=[]  NTsProdOutMax=[]  UintegralTsProdOutMin=[]  UintegralTsProdOutMax=[]  UngainTsProdOutMin=[]  UngainTsProdOutMax=[]  ClampingZeroOutDataTypeStr=Inherit: Inherit via back propagation  ClampingZeroOutMin=[]  ClampingZeroOutMax=[]  FilterDenConstantOutDataTypeStr=Inherit: Inherit via back propagation  FilterDenConstantOutMin=[]  FilterDenConstantOutMax=[]  PCopyOutDataTypeStr=Inherit: Inherit via back propagation  PCopyOutMin=[]  PCopyOutMax=[]  NCopyOutDataTypeStr=Inherit: Inherit via back propagation  NCopyOutMin=[]  NCopyOutMax=[]  IntegratorContinuousStateAttributes=''  IntegratorStateMustResolveToSignalObject=off  IntegratorRTWStateStorageClass=Auto  FilterContinuousStateAttributes=''  FilterStateMustResolveToSignalObject=off  FilterRTWStateStorageClass=Auto  ParallelPVariant=InternalParameters  IdealPVariant=Disabled  IVariant=InternalParameters  DVariant=InternalParameters  IntegratorVariant=Continuous  SatVariant=Disabled  AWVariant=Passthrough  PCopyVariant=Disabled  TRVariant=Disabled  FdbkBlocksVariant=Forward  IdealPFdbkVariant=Disabled  SatFdbkVariant=Disabled  DerivativeFilterVariant=ContFilter  NVariant=InternalParameters  NCopyVariant=Disabled  FilterICVariant=InternalICsFilter  IntegratorICVariant=InternalICs  ExternalResetVariant=Disabled  TRSumVariant=Passthrough  SumFdbkVariant=Disabled  SumVariant=Sum_PID  TsampFilterVariant=InternalTs  TsampNgainVariant=Passthrough  TsampIntegralVariant=Disabled_SignalSpec  ExternalSaturationOutDataTypeStr=Inherit: Same as second input  DerivativeSourceVariant=ErrorSignal
  PLL (3ph) : spsPLL3phLib/PLL (3ph)  Fmin=45  Par_Init=[0, 60]  ParK=[180, 3200, 1]  TcD=1e-4  MaxRateChangeFreq=12  FilterCutOffFreq=25  Ts=0  AGC=on
  abc to dq0 : spsabctodq0Lib/abc to dq0  Alignment=90 degrees behind phase A axis
  abc to dq1 : spsabctodq0Lib/abc to dq0  Alignment=90 degrees behind phase A axis
  dq0 to abc : spsdq0toabcLib/dq0 to abc  Alignment=90 degrees behind phase A axis
  Vabc_c : Outport
  tag scope: Id=global, Id_ref=global, Iq=global, Vd_control=global, Vd_in=global, Vq_control=global, Vq_in=global, null1=global, null2=global
  wires:
  Demux1/1 -> [Id]
  Add2/1 -> PID Controller1/1
  [Vd_control] -> Mux/1
  [Id_ref] -> Add1/2
  Iabc/1 -> abc to dq0/1
  [Iq] -> Gain1/1, Add2/1
  PLL (3ph)/1 -> [null2]
  Vabc/1 -> abc to dq1/1, PLL (3ph)/1
  [Id] -> Gain2/1, Add1/1
  abc to dq0/1 -> Demux1/1
  Add3/1 -> [Vd_control]
  Demux1/2 -> [Iq]
  [Vq_control] -> Mux/2
  Iq_ref/1 -> Add2/2
  Demux1/3 -> [null1]
  Iq_ref1/1 -> Mux/3
  Add4/1 -> [Vq_control]
  PLL (3ph)/2 -> [Wt], abc to dq0/2
  Mux/1 -> dq0 to abc/1
  Add1/1 -> PID Controller3/1
  Gain1/1 -> Add3/2
  abc to dq1/1 -> Demux2/1
  Demux2/1 -> [Vd_in]
  Demux2/2 -> [Vq_in]
  [Vd_in] -> Add3/3
  Gain2/1 -> Add4/2
  [Vq_in] -> Add4/3
  dq0 to abc/1 -> Vabc_c/1
  PID Controller3/1 -> Add3/1
  PID Controller1/1 -> Add4/1
  [Wt] -> dq0 to abc/2
  [Wt] -> abc to dq1/2
  PID Controller2/1 -> [Id_ref]
  Vdc/1 -> Add/1
  Vref/1 -> Add/2
  Add/1 -> PID Controller2/1

== matlab function SYSTEM_MODEL/control/MATLAB Function ==
  data: SOC input; state output
function state = fcn(SOC)
%#codegen

persistent prev_state
if isempty(prev_state)
    prev_state = 0;   % 0 = CC, 1 = CV
end

if SOC >= 80
    state = 0;        % CV
elseif SOC < 80
    state = 1;        % CC
else
    state = prev_state;
end

prev_state = state;

== matlab function SYSTEM_MODEL/Coolant pump flow ==
  data: Tbat input; pump_flow output
function pump_flow = Pump(Tbat)

if Tbat > 50
    pump_flow = 1; % full cooling
elseif Tbat < 30
    pump_flow = 0.2; % minimal cooling
else
    pump_flow = 0.5; % moderate
end

== matlab function SYSTEM_MODEL/Battery module/MATLAB Function ==
  data: Ibat input; Tbat output; pump_flow input; Tcool output
function [Tbat, Tcool] = battery_liquid_cooling(Ibat, pump_flow)
%#codegen
% Signal-based battery + glycol-water cooling model
% Inputs:
%   Ibat       - battery current [A]
%   pump_flow  - 0 to 1, fraction of coolant flow rate
% Outputs:
%   Tbat       - battery temperature [°C]
%   Tcool      - coolant temperature [°C]

persistent T_b T_c
if isempty(T_b)
    T_b = 25;   % Initial battery temp (°C)
    T_c = 20;   % Initial coolant temp (°C)
end



% --- Parameters ---
R_int   = 0.05;       % Battery internal resistance [Ohm]
Cth_b   = 500*1000;    % Battery thermal mass [J/°C]
Cth_c   = 500;         % Coolant lumped thermal mass [J/°C]
hA      = 50*3;        % Heat transfer W/°C (h*A)
T_cool  = 20;          % Coolant inlet temp
Ts      = 3e-6;        % Simulation timestep
Tamb = 25;              % Ambient temperature (°C)
hA_amb = 5 * 3;         % Air convection (W/°C), low value

Qamb = hA_amb * (T_b - Tamb);


% --- Battery heat generation ---
Qgen = Ibat^2 * R_int;

% --- Heat transfer to coolant ---
Qcool = hA * (T_b - T_c) * pump_flow;

% --- Battery temperature update ---
%dT_b = (Qgen - Qcool)/Cth_b;
dT_b = (Qgen - Qcool - Qamb)/Cth_b;

T_b = T_b + Ts*dT_b;

% --- Coolant temperature update ---
dT_c = (Qcool + 0)/Cth_c;  % 0 = no ambient heat loss for simplicity
T_c = T_c + Ts*dT_c;

% --- Output ---
Tbat = T_b;
Tcool = T_c;
